simulink model "elp_watchdog_reset"  (R2026b)
settings: Solver=VariableStepAuto
undefined symbols (not defined in the file or in its folder): P, Ts
libraries: simulink x5
settings Model: Creator=aomar  LastModifiedBy=aomar

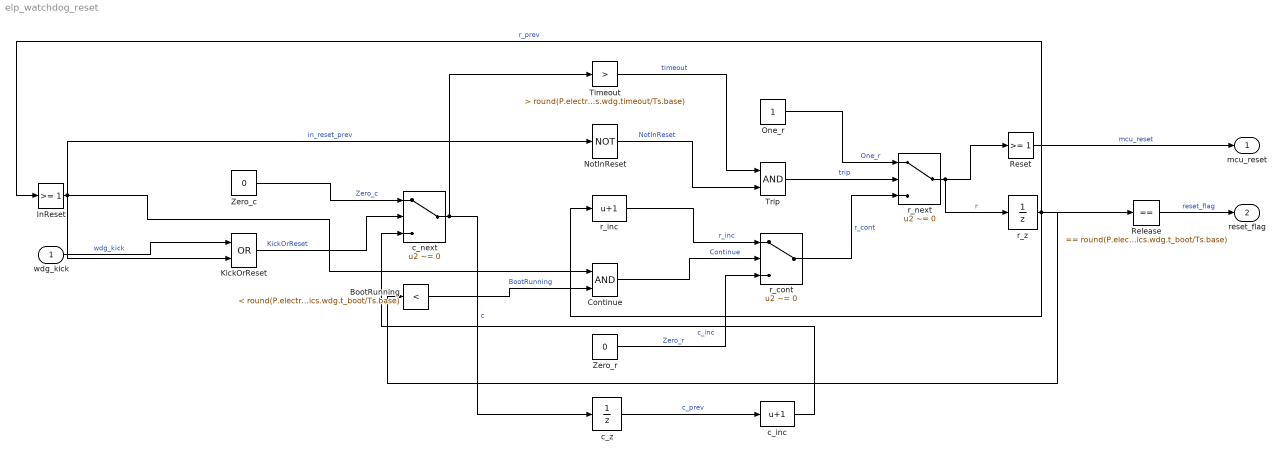
== system elp_watchdog_reset ==
  wdg_kick : Inport  OutDataTypeStr=boolean  SampleTime=Ts.base
  BootRunning : simulink/Logic and Bit Operations/Compare To Constant  relop=<  const=round(P.electronics.wdg.t_boot/Ts.base)  OutDataTypeStr=boolean
  Continue : Logic  AllPortsSameDT=off  OutDataTypeStr=boolean
  InReset : simulink/Logic and Bit Operations/Compare To Constant  relop=>=  const=1  OutDataTypeStr=boolean
  KickOrReset : Logic  Operator=OR  AllPortsSameDT=off  OutDataTypeStr=boolean
  NotInReset : Logic  Operator=NOT  Inputs=1  AllPortsSameDT=off  OutDataTypeStr=boolean
  One_r : Constant  OutDataTypeStr=double  SampleTime=Ts.base
  Release : simulink/Logic and Bit Operations/Compare To Constant  relop===  const=round(P.electronics.wdg.t_boot/Ts.base)  OutDataTypeStr=boolean
  Reset : simulink/Logic and Bit Operations/Compare To Constant  relop=>=  const=1  OutDataTypeStr=boolean
  Timeout : simulink/Logic and Bit Operations/Compare To Constant  relop=>  const=round(P.electronics.wdg.timeout/Ts.base)  OutDataTypeStr=boolean
  Trip : Logic  AllPortsSameDT=off  OutDataTypeStr=boolean
  Zero_c : Constant  Value=0  OutDataTypeStr=double  SampleTime=Ts.base
  Zero_r : Constant  Value=0  OutDataTypeStr=double  SampleTime=Ts.base
  c_inc : Bias  Bias=1  SaturateOnIntegerOverflow=off
  c_next : Switch  Criteria=u2 ~= 0  SaturateOnIntegerOverflow=off  InputSameDT=off
  c_z : UnitDelay  SampleTime=Ts.base
  r_cont : Switch  Criteria=u2 ~= 0  SaturateOnIntegerOverflow=off  InputSameDT=off
  r_inc : Bias  Bias=1  SaturateOnIntegerOverflow=off
  r_next : Switch  Criteria=u2 ~= 0  SaturateOnIntegerOverflow=off  InputSameDT=off
  r_z : UnitDelay  SampleTime=Ts.base
  mcu_reset : Outport  OutDataTypeStr=boolean
  reset_flag : Outport  Port=2  OutDataTypeStr=boolean
  wires:
  InReset/1 -> Continue/1, KickOrReset/2, NotInReset/1  "in_reset_prev"
  wdg_kick/1 -> KickOrReset/1  "wdg_kick"
  Zero_c/1 -> c_next/1  "Zero_c"
  KickOrReset/1 -> c_next/2  "KickOrReset"
  BootRunning/1 -> Continue/2  "BootRunning"
  c_next/1 -> c_z/1, Timeout/1  "c"
  Timeout/1 -> Trip/1  "timeout"
  NotInReset/1 -> Trip/2  "NotInReset"
  Continue/1 -> r_cont/2  "Continue"
  Zero_r/1 -> r_cont/3  "Zero_r"
  c_z/1 -> c_inc/1  "c_prev"
  r_inc/1 -> r_cont/1  "r_inc"
  One_r/1 -> r_next/1  "One_r"
  Trip/1 -> r_next/2  "trip"
  c_inc/1 -> c_next/3  "c_inc"
  r_cont/1 -> r_next/3  "r_cont"
  r_next/1 -> Reset/1, r_z/1  "r"
  Reset/1 -> mcu_reset/1  "mcu_reset"
  r_z/1 -> BootRunning/1, InReset/1, r_inc/1, Release/1  "r_prev"
  Release/1 -> reset_flag/1  "reset_flag"
